simulink model "A3_5_tilt"  (R2024b)
settings: Solver=ode4  StartTime=0.0  StopTime=T_run  FixedStep=Ts_ctrl  RelTol=1e-3
InitFcn:
  | if ~exist('A3_model_init','file'), addpath(fileparts(get_param('A3_5_tilt','FileName'))); end, A3_model_init('A3_5_tilt')
StopFcn:
  | A3_model_done('A3_5_tilt')
values from neighbouring files (symbols this model uses):
  d_max = 45*pi/180    (= 0.785398163397)    [A3_azpolar_example.m]    (also in A3_nullspace_example.m; A3_pinv_example.m; A3_setup.m = deg2rad(d_max_deg))
  svo_rate = deg2rad(svo_rate_deg)    [A3_setup.m]
  svo_tau = svo_tau_s    (= 0.2)    [A3_setup.m]
  tilt_q = [tilt_hold; tilt_thrust; size(tilt_deg,1);            reshape(deg2rad(tilt_deg)', [], 1)]    [A3_setup.m]
  Ts_ctrl = 0.05    [A3_setup.m]
  vrx_pos_sign = -1    [A3_setup.m]
libraries: ros2lib x8
settings Model: Creator=admin  LastModifiedBy=admin

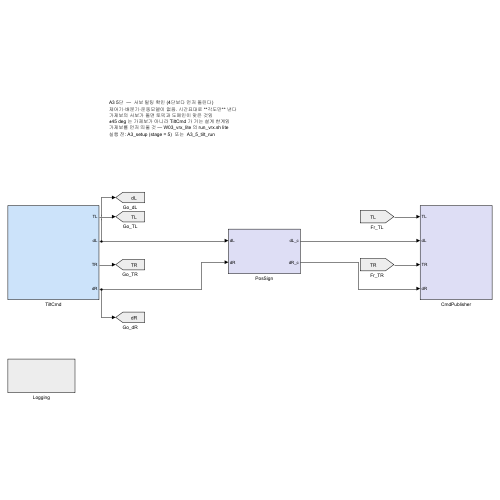
[thumbnail: Simulink's stored preview of the top-level diagram]
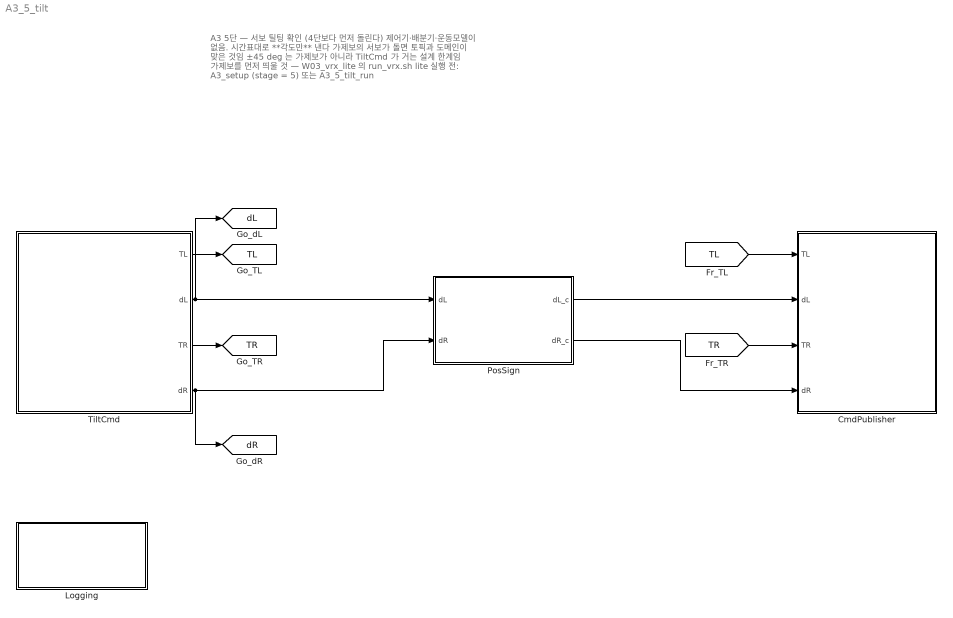
== system A3_5_tilt ==
  note: A3 5단  —  서보 틸팅 확인 (4단보다 먼저 돌린다)
      | 제어기·배분기·운동모델이 없음. 시간표대로 **각도만** 낸다
      | 가제보의 서보가 돌면 토픽과 도메인이 맞은 것임
      | ±45 deg 는 가제보가 아니라 TiltCmd 가 거는 설계 한계임
      | 가제보를 먼저 띄울 것 — W03_vrx_lite 의 run_vrx.sh lite
      | 실행 전: A3_setup (stage = 5)  또는  A3_5_tilt_run
  CmdPublisher : Subsystem
  Logging : Subsystem
  PosSign : Subsystem
  TiltCmd : Subsystem
  tag scope: TL=global, TR=global, dL=global, dR=global
  wires:
  PosSign/2(dR_c) -> CmdPublisher/4(dR)
  PosSign/1(dL_c) -> CmdPublisher/2(dL)
  TiltCmd/4(dR) -> PosSign/2(dR), [dR]
  TiltCmd/2(dL) -> PosSign/1(dL), [dL]
  TiltCmd/1(TL) -> [TL]
  TiltCmd/3(TR) -> [TR]
  [TL] -> CmdPublisher/1(TL)
  [TR] -> CmdPublisher/3(TR)

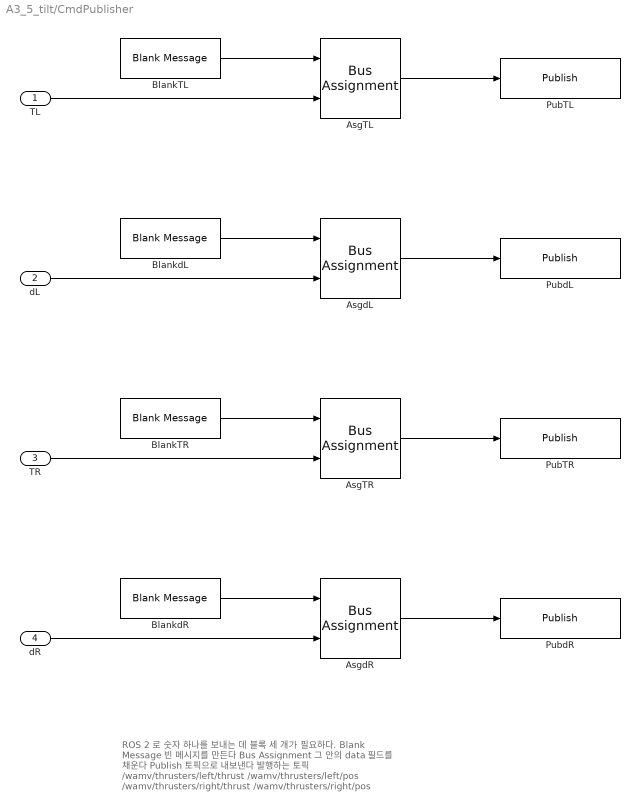
== system A3_5_tilt/CmdPublisher ==
  note: ROS 2 로 숫자 하나를 보내는 데 블록 세 개가 필요하다.
      |   Blank Message   빈 메시지를 만든다
      |   Bus Assignment  그 안의 data 필드를 채운다
      |   Publish         토픽으로 내보낸다
      |
      | 발행하는 토픽
      | /wamv/thrusters/left/thrust
      | /wamv/thrusters/left/pos
      | /wamv/thrusters/right/thrust
      | /wamv/thrusters/right/pos
  TL : Inport
  dL : Inport  Port=2
  TR : Inport  Port=3
  dR : Inport  Port=4
  AsgTL : BusAssignment  AssignedSignals=data
  AsgTR : BusAssignment  AssignedSignals=data
  AsgdL : BusAssignment  AssignedSignals=data
  AsgdR : BusAssignment  AssignedSignals=data
  BlankTL : ros2lib/Blank Message  messageClass=Message  entityType=std_msgs/Float64  messageType=std_msgs/Float64  SampleTime=Ts_ctrl
  BlankTR : ros2lib/Blank Message  messageClass=Message  entityType=std_msgs/Float64  messageType=std_msgs/Float64  SampleTime=Ts_ctrl
  BlankdL : ros2lib/Blank Message  messageClass=Message  entityType=std_msgs/Float64  messageType=std_msgs/Float64  SampleTime=Ts_ctrl
  BlankdR : ros2lib/Blank Message  messageClass=Message  entityType=std_msgs/Float64  messageType=std_msgs/Float64  SampleTime=Ts_ctrl
  PubTL : ros2lib/Publish  topicSource=Specify your own  topic=/wamv/thrusters/left/thrust  messageType=std_msgs/Float64  QOSHistory=Keep last  QOSDepth=1  QOSReliability=Reliable  QOSDurability=Volatile  QOSDeadline=Inf  QOSLifespan=Inf  QOSLiveliness=Automatic  QOSLeaseDuration=Inf  QOSAvoidROSNamespaceConventions=off
  PubTR : ros2lib/Publish  topicSource=Specify your own  topic=/wamv/thrusters/right/thrust  messageType=std_msgs/Float64  QOSHistory=Keep last  QOSDepth=1  QOSReliability=Reliable  QOSDurability=Volatile  QOSDeadline=Inf  QOSLifespan=Inf  QOSLiveliness=Automatic  QOSLeaseDuration=Inf  QOSAvoidROSNamespaceConventions=off
  PubdL : ros2lib/Publish  topicSource=Specify your own  topic=/wamv/thrusters/left/pos  messageType=std_msgs/Float64  QOSHistory=Keep last  QOSDepth=1  QOSReliability=Reliable  QOSDurability=Volatile  QOSDeadline=Inf  QOSLifespan=Inf  QOSLiveliness=Automatic  QOSLeaseDuration=Inf  QOSAvoidROSNamespaceConventions=off
  PubdR : ros2lib/Publish  topicSource=Specify your own  topic=/wamv/thrusters/right/pos  messageType=std_msgs/Float64  QOSHistory=Keep last  QOSDepth=1  QOSReliability=Reliable  QOSDurability=Volatile  QOSDeadline=Inf  QOSLifespan=Inf  QOSLiveliness=Automatic  QOSLeaseDuration=Inf  QOSAvoidROSNamespaceConventions=off
  wires:
  BlankTL/1 -> AsgTL/1
  AsgTL/1 -> PubTL/1
  TL/1 -> AsgTL/2
  BlankdL/1 -> AsgdL/1
  AsgdL/1 -> PubdL/1
  dL/1 -> AsgdL/2
  BlankTR/1 -> AsgTR/1
  AsgTR/1 -> PubTR/1
  TR/1 -> AsgTR/2
  BlankdR/1 -> AsgdR/1
  AsgdR/1 -> PubdR/1
  dR/1 -> AsgdR/2

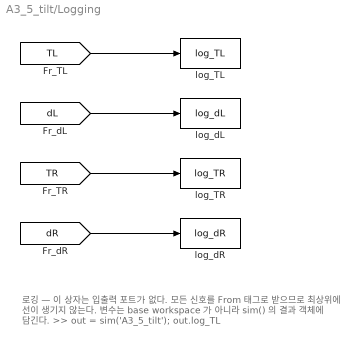
== system A3_5_tilt/Logging ==
  note: 로깅 — 이 상자는 입출력 포트가 없다.
      | 모든 신호를 From 태그로 받으므로 최상위에 선이 생기지 않는다.
      | 변수는 base workspace 가 아니라 sim() 의 결과 객체에 담긴다.
      |   >> out = sim('A3_5_tilt');  out.log_TL
  log_TL : ToWorkspace  VariableName=log_TL  SaveFormat=Timeseries  SampleTime=Ts_ctrl
  log_TR : ToWorkspace  VariableName=log_TR  SaveFormat=Timeseries  SampleTime=Ts_ctrl
  log_dL : ToWorkspace  VariableName=log_dL  SaveFormat=Timeseries  SampleTime=Ts_ctrl
  log_dR : ToWorkspace  VariableName=log_dR  SaveFormat=Timeseries  SampleTime=Ts_ctrl
  wires:
  [TL] -> log_TL/1
  [dL] -> log_dL/1
  [TR] -> log_TR/1
  [dR] -> log_dR/1

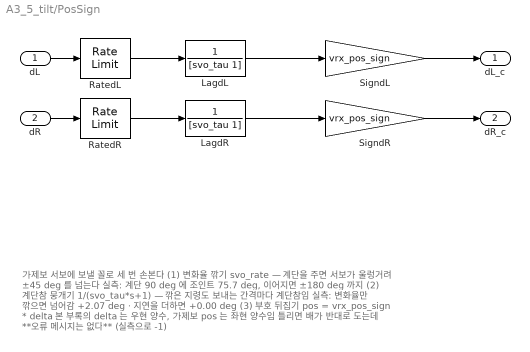
== system A3_5_tilt/PosSign ==
  note: 가제보 서보에 보낼 꼴로 세 번 손본다
      | (1) 변화율 깎기 svo_rate — 계단을 주면 서보가 울렁거려 ±45 deg 를 넘는다
      |       실측: 계단 90 deg 에 조인트 75.7 deg, 이어지면 ±180 deg 까지
      | (2) 계단참 뭉개기 1/(svo_tau*s+1) — 깎은 지령도 보내는 간격마다 계단참임
      |       실측: 변화율만 깎으면 넘어감 +2.07 deg · 지연을 더하면 +0.00 deg
      | (3) 부호 뒤집기 pos = vrx_pos_sign * delta
      |       본 부록의 delta 는 우현 양수, 가제보 pos 는 좌현 양수임
      |       틀리면 배가 반대로 도는데 **오류 메시지는 없다** (실측으로 -1)
  dL : Inport
  dR : Inport  Port=2
  LagdL : TransferFcn  Denominator=[svo_tau 1]
  LagdR : TransferFcn  Denominator=[svo_tau 1]
  RatedL : RateLimiter  RisingSlewLimit=svo_rate  FallingSlewLimit=-svo_rate  SampleTimeMode=inherited
  RatedR : RateLimiter  RisingSlewLimit=svo_rate  FallingSlewLimit=-svo_rate  SampleTimeMode=inherited
  SigndL : Gain  Gain=vrx_pos_sign
  SigndR : Gain  Gain=vrx_pos_sign
  dL_c : Outport
  dR_c : Outport  Port=2
  wires:
  dL/1 -> RatedL/1
  RatedL/1 -> LagdL/1
  LagdL/1 -> SigndL/1
  SigndL/1 -> dL_c/1
  dR/1 -> RatedR/1
  RatedR/1 -> LagdR/1
  LagdR/1 -> SigndR/1
  SigndR/1 -> dR_c/1

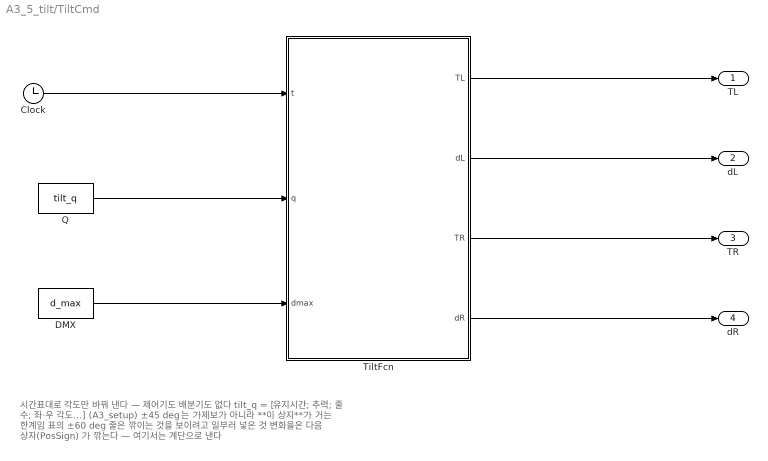
== system A3_5_tilt/TiltCmd ==
  note: 시간표대로 각도만 바꿔 낸다 — 제어기도 배분기도 없다
      | tilt_q = [유지시간; 추력; 줄 수; 좌·우 각도...]  (A3_setup)
      | ±45 deg 는 가제보가 아니라 **이 상자**가 거는 한계임
      | 표의 ±60 deg 줄은 깎이는 것을 보이려고 일부러 넣은 것
      | 변화율은 다음 상자(PosSign) 가 깎는다 — 여기서는 계단으로 낸다
  Clock : Clock
  DMX : Constant  Value=d_max
  Q : Constant  Value=tilt_q
  TiltFcn : MATLAB Function  TreatAsAtomicUnit=on
  TL : Outport
  dL : Outport  Port=2
  TR : Outport  Port=3
  dR : Outport  Port=4
  wires:
  Clock/1 -> TiltFcn/1(t)
  Q/1 -> TiltFcn/2(q)
  DMX/1 -> TiltFcn/3(dmax)
  TiltFcn/1(TL) -> TL/1
  TiltFcn/2(dL) -> dL/1
  TiltFcn/4(dR) -> dR/1
  TiltFcn/3(TR) -> TR/1

== matlab function A3_5_tilt/TiltCmd/TiltFcn ==
  data: t input; TL output; q input; dmax input; dL output; TR output; dR output
function [TL, dL, TR, dR] = TiltFcn(t, q, dmax)
%#codegen
%  시간표대로 방향각을 내는 함수 — 추력은 상수, 각도만 바뀐다
%    q(1)        한 자세를 유지하는 시간 [s]
%    q(2)        그 동안 줄 추력 [N]
%    q(3)        표의 줄 수 n
%    q(4:3+2n)   [좌현; 우현] 각도가 줄 순서대로 [rad]

hold_t = q(1);
T_cmd  = q(2);
n      = q(3);

%  몇 번째 줄인가 — 마지막 줄을 지나면 그 줄에 머문다 (중립으로 끝난다)
i = floor(t/hold_t) + 1;
if i < 1, i = 1; end
if i > n, i = n; end

%  q 안에서 그 줄이 시작하는 자리. 줄 하나가 두 칸을 쓴다
j  = 3 + 2*(i-1);
dL = q(j+1);
dR = q(j+2);

%  **설계 한계** — 가제보 조인트에는 없는 한계를 여기서 건다
%    표의 ±60 deg 줄이 ±45 deg 로 깎이는 것이 이 두 줄이다
dL = max(min(dL, dmax), -dmax);
dR = max(min(dR, dmax), -dmax);

TL = T_cmd;
TR = T_cmd;
end
